simulink model "realimentacion_observador"  (R2018a)
settings: Solver=VariableStepAuto  StartTime=0.0  StopTime=50  RelTol=1e-3
undefined symbols (not defined in the file): den_c, den_p, num_c, num_p
settings Model: Creator=Karel  LastModifiedBy=Karel

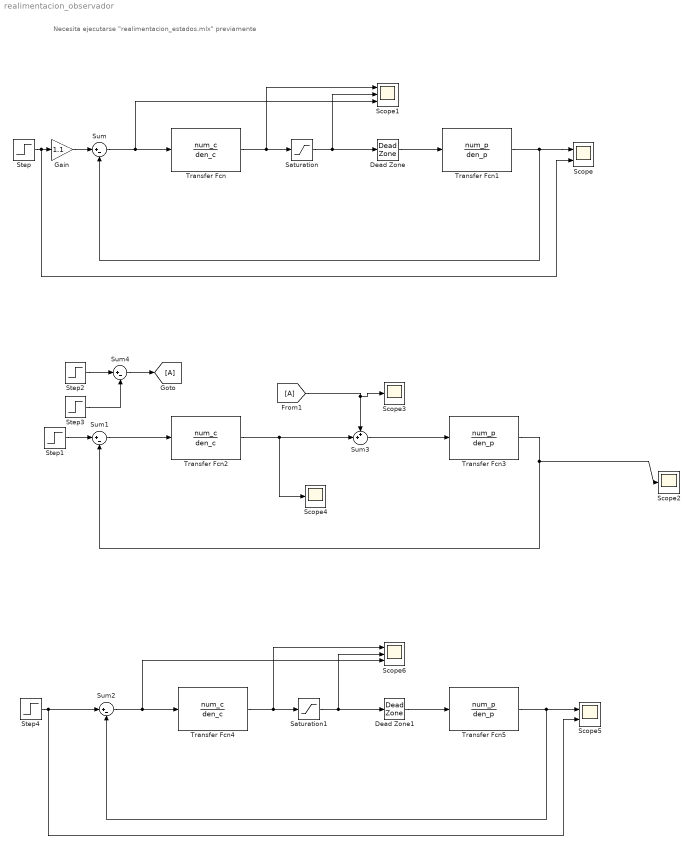
== system realimentacion_observador ==
  note: Necesita ejecutarse "realimentacion_estados.mlx" previamente
  Dead Zone : DeadZone  LowerValue=0  UpperValue=0.2  SaturateOnIntegerOverflow=on
  Dead Zone1 : DeadZone  LowerValue=0  UpperValue=0.2  SaturateOnIntegerOverflow=on
  Gain : Gain  Gain=1.1
  Saturation : Saturate  UpperLimit=10  LowerLimit=0
  Saturation1 : Saturate  UpperLimit=10  LowerLimit=0
  Scope : Scope  NumInputPorts=2
  Scope1 : Scope  NumInputPorts=3
  Scope2 : Scope
  Scope3 : Scope
  Scope4 : Scope
  Scope5 : Scope  NumInputPorts=2
  Scope6 : Scope  NumInputPorts=3
  Step : Step  After=10  SampleTime=0
  Step1 : Step  After=360  SampleTime=0
  Step2 : Step  Time=7  After=3  SampleTime=0
  Step3 : Step  Time=7.1  After=3  SampleTime=0
  Step4 : Step  After=10  SampleTime=0
  Sum{,1..2,4} (4 alike) : Sum  Inputs=|+-
  Sum3 : Sum  Inputs=++|
  Transfer Fcn : TransferFcn  Numerator=num_c  Denominator=den_c
  Transfer Fcn1 : TransferFcn  Numerator=num_p  Denominator=den_p
  Transfer Fcn2 : TransferFcn  Numerator=num_c  Denominator=den_c
  Transfer Fcn3 : TransferFcn  Numerator=num_p  Denominator=den_p
  Transfer Fcn4 : TransferFcn  Numerator=num_c  Denominator=den_c
  Transfer Fcn5 : TransferFcn  Numerator=num_p  Denominator=den_p
  wires:
  Transfer Fcn/1 -> Saturation/1, Scope1/1
  Transfer Fcn1/1 -> Scope/1, Sum/2
  Sum/1 -> Scope1/3, Transfer Fcn/1
  Step1/1 -> Sum1/1
  Sum1/1 -> Transfer Fcn2/1
  Transfer Fcn3/1 -> Scope2/1, Sum1/2
  Transfer Fcn2/1 -> Scope4/1, Sum3/2
  Sum3/1 -> Transfer Fcn3/1
  [A] -> Scope3/1, Sum3/1
  Step2/1 -> Sum4/1
  Sum4/1 -> [A]
  Step3/1 -> Sum4/2
  Saturation/1 -> Dead Zone/1, Scope1/2
  Dead Zone/1 -> Transfer Fcn1/1
  Gain/1 -> Sum/1
  Step/1 -> Scope/2, Gain/1
  Step4/1 -> Sum2/1, Scope5/2
  Dead Zone1/1 -> Transfer Fcn5/1
  Saturation1/1 -> Scope6/2, Dead Zone1/1
  Sum2/1 -> Transfer Fcn4/1, Scope6/3
  Transfer Fcn5/1 -> Sum2/2, Scope5/1
  Transfer Fcn4/1 -> Scope6/1, Saturation1/1
